simulink model "CSTR_Simulink"  (R2026a)
settings: Solver=ode15s  StopTime=model.time  FixedStep=5./60./10000
values from neighbouring files (symbols this model uses):
  A = 16.66    [plant_data_gen.m]
  Cv_Q = SS.Q ./ ( SS.lQ .* N .* sqrt( ( SS.P_U - SS.P_D ) ./ g_s) )    [plant_data_gen.m]
  Cv_Q_C = SS.Q_C ./ ( SS.lQ_C .* N .* sqrt( ( SS.P_CU - SS.P_CD ) ./ g_s ) )    [plant_data_gen.m]
  deltaH = -5e4    (= -50000)    [plant_data_gen.m]
  EoR = 8750    [plant_data_gen.m]
  g_s = 1    [plant_data_gen.m]
  K = size(x)    [PPCA_validation.m]    (also in plant_data_gen.m = 0.0625)
  k_0 = 7.2e10    (= 72000000000)    [plant_data_gen.m]
  Kc_h = -3.0    (= -3)    [plant_data_gen.m]
  Kc_Q = 0.2    [plant_data_gen.m]
  Kc_Q_C = 0.2    [plant_data_gen.m]
  Kc_T = -2.0    (= -2)    [plant_data_gen.m]
  Km_Q = 8/100    (= 0.08)    [plant_data_gen.m]
  Km_Q_C = 8/15    (= 0.533333333333)    [plant_data_gen.m]
  N = 0.0865 * 1000 / 60 / sqrt(1000)    [plant_data_gen.m]
  rhoCp = 239    [plant_data_gen.m]
  rhoCp_C = 4175    [plant_data_gen.m]
  tau = 2./60    (= 0.0333333333333)    [plant_data_gen.m]
  TI_h = 1./TI_h    (= 0.666666666667)    [plant_data_gen.m]
  TI_Q = 1.7/60    (= 0.0283333333333)    [plant_data_gen.m]
  TI_Q_C = 1./TI_Q_C    (= 35.2941176471)    [plant_data_gen.m]
  TI_T = 1./TI_T    (= 1.14942528736)    [plant_data_gen.m]
  UA_C = 5e4    (= 50000)    [plant_data_gen.m]
  V_C = 10    [plant_data_gen.m]
undefined symbols (not defined in the file or in its folder): D, model, noise, SS
libraries: dspsrcs4 x16, simulink x8, slpidlib x4
(part 1 of 2)
settings Model: Creator=danie  LastModifiedBy=daniel

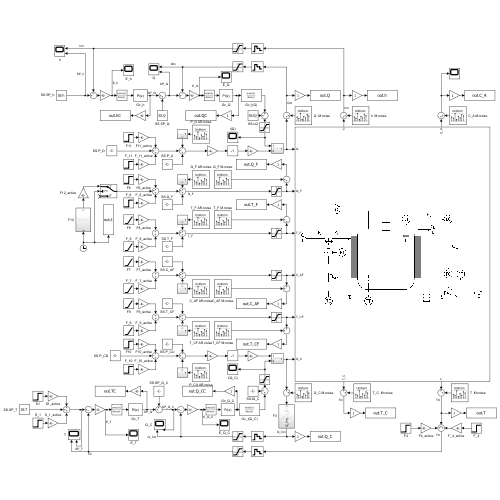
[thumbnail: Simulink's stored preview of the top-level diagram]
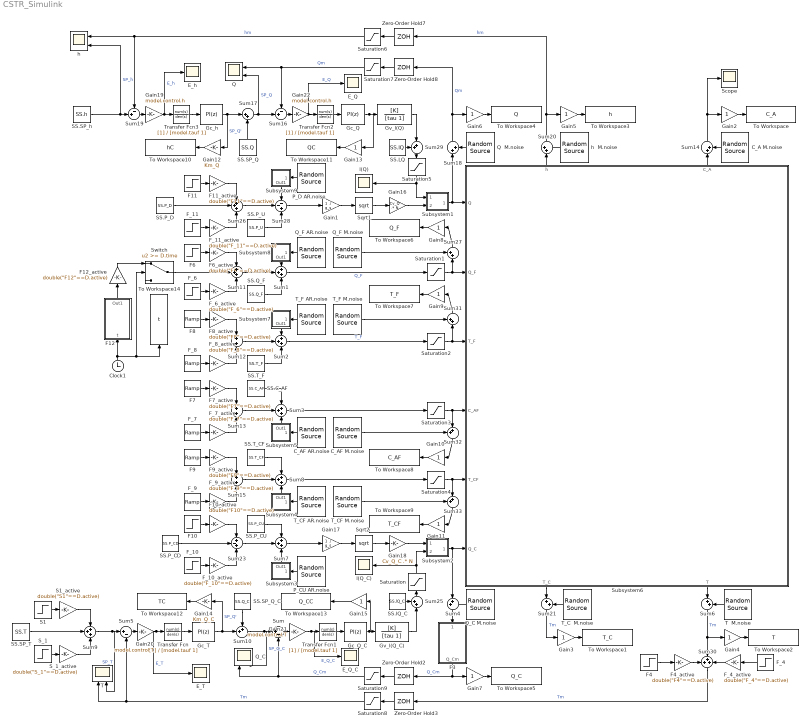
== system CSTR_Simulink ==
  C_A M.noise : dspsrcs4/Random Source  SrcType=Gaussian  MinVal=0  MaxVal=1  MeanVal=0  VarVal=noise.M.C_A.*noise.M.active  RepMode=Not repeatable  rawSeed=5  IsInherit=off  SampTime=model.dt  SampFrame=1  OutComplex=Real  DataType=double  SimulateUsing=Interpreted execution
  C_AF AR.noise : dspsrcs4/Random Source  SrcType=Gaussian  MinVal=0  MaxVal=1  MeanVal=0  VarVal=noise.AR.C_AF.*noise.AR.active  RepMode=Not repeatable  rawSeed=736  IsInherit=off  SampTime=model.dt  SampFrame=1  OutComplex=Real  DataType=double  SimulateUsing=Interpreted execution
  C_AF M.noise : dspsrcs4/Random Source  SrcType=Gaussian  MinVal=0  MaxVal=1  MeanVal=0  VarVal=noise.M.C_AF.*noise.M.active  RepMode=Not repeatable  rawSeed=3456  IsInherit=off  SampTime=model.dt  SampFrame=1  OutComplex=Real  DataType=double  SimulateUsing=Interpreted execution
  Clock1 : Clock
  E_Q : Scope
      settings: ActiveDisplayYMinimum=-115  ActiveDisplayYMaximum=135  DataLoggingVariableName=ScopeData6
  E_Q_C : Scope
      settings: ActiveDisplayYMinimum=-0.48410226680583923  ActiveDisplayYMaximum=0.37217378043200133  DataLoggingVariableName=ScopeData5
  E_T : Scope
      settings: ActiveDisplayYMinimum=-14.355250634138558  ActiveDisplayYMaximum=1.5950278482376172  DataLoggingVariableName=ScopeData4
  E_h : Scope
      settings: ActiveDisplayYMinimum=-14.355250634138558  ActiveDisplayYMaximum=1.5950278482376172  DataLoggingVariableName=ScopeData7
  F{4,6,10..11} (4 alike) : Step  Time=D.time  FinalValue=D.val  SampleTime=0
  F10_active : Gain  Gain="double(\"F10\"==D.active)"
  F11_active : Gain  Gain="double(\"F11\"==D.active)"
  F12 : Subsystem
  F12_active : Gain  Gain="double(\"F12\"==D.active)"
  F3 : Subsystem
  F4_active : Gain  Gain="double(\"F4\"==D.active)"
  F6_active : Gain  Gain="double(\"F6\"==D.active)"
  F7 : simulink/Sources/Ramp  slope=D.val  start=D.time  InitialOutput=0
  F7_active : Gain  Gain="double(\"F7\"==D.active)"
  F8 : simulink/Sources/Ramp  slope=D.val  start=D.time  InitialOutput=0
  F8_active : Gain  Gain="double(\"F8\"==D.active)"
  F9 : simulink/Sources/Ramp  slope=D.val  start=D.time  InitialOutput=0
  F9_active : Gain  Gain="double(\"F9\"==D.active)"
  F_{4,6,10..11} (4 alike) : Step  Time=D.time  FinalValue=D.val  SampleTime=0
  F_10_active : Gain  Gain="double(\"F_10\"==D.active)"
  F_11_active : Gain  Gain="double(\"F_11\"==D.active)"
  F_4_active : Gain  Gain="double(\"F_4\"==D.active)"
  F_6_active : Gain  Gain="double(\"F_6\"==D.active)"
  F_7 : simulink/Sources/Ramp  slope=D.val  start=D.time  InitialOutput=0
  F_7_active : Gain  Gain="double(\"F_7\"==D.active)"
  F_8 : simulink/Sources/Ramp  slope=D.val  start=D.time  InitialOutput=0
  F_8_active : Gain  Gain="double(\"F_8\"==D.active)"
  F_9 : simulink/Sources/Ramp  slope=D.val  start=D.time  InitialOutput=0
  F_9_active : Gain  Gain="double(\"F_9\"==D.active)"
  Gain1 : Gain  Gain=1 ./ g_s
  Gain{2..11,13,15} (12 alike) : Gain
  Gain12 : Gain  Gain=Km_Q
  Gain14 : Gain  Gain=Km_Q_C
  Gain16 : Gain  Gain=Cv_Q .* N
  Gain17 : Gain  Gain=1 ./ g_s
  Gain18 : Gain  Gain=Cv_Q_C .* N
  Gain19 : Gain  Gain=model.control.h
  Gain20 : Gain  Gain=model.control.T
  Gain21 : Gain  Gain=model.control.T
  Gain22 : Gain  Gain=model.control.h
  Gc_Q : slpidlib/PID Controller  Controller=PI  Form=Ideal  TimeDomain=Discrete-time  UseExternalTs=off  SampleTime=model.dt  IntegratorMethod=Forward Euler  FilterMethod=Forward Euler  ControllerParametersSource=internal  P=Kc_Q  I=TI_Q  UseKiTs=off  D=0  UseExternalDerivativeSource=off  N=100  UseFilter=on  TunerSelectOption=Transfer Function Based (PID Tuner App)  InitialConditionSource=internal  InitialConditionForIntegrator=0  InitialConditionForFilter=0  DifferentiatorICPrevScaledInput=0  ExternalReset=none  TrackingMode=off  Kt=1  LimitOutput=off  SatLimitsSource=internal  UpperSaturationLimit=inf  LowerSaturationLimit=-inf  LinearizeAsGain=on  AntiWindupMode=none  Kb=1  LimitIntegrator=off  UpperIntegratorSaturationLimit=inf  LowerIntegratorSaturationLimit=-inf  POutMin=[]  POutMax=[]  IOutMin=[]  IOutMax=[]  DOutMin=[]  DOutMax=[]  NOutMin=[]  NOutMax=[]  SumOutMin=[]  SumOutMax=[]  SaturationOutMin=[]  SaturationOutMax=[]  PParamMin=[]  PParamMax=[]  IParamMin=[]  IParamMax=[]  DParamMin=[]  DParamMax=[]  NParamMin=[]  NParamMax=[]  KbParamMin=[]  KbParamMax=[]  KtParamMin=[]  KtParamMax=[]  KbOutMin=[]  KbOutMax=[]  KtOutMin=[]  KtOutMax=[]  IntegratorOutMin=[]  IntegratorOutMax=[]  FilterOutMin=[]  FilterOutMax=[]  SumI1OutMin=[]  SumI1OutMax=[]  SumI2OutMin=[]  SumI2OutMax=[]  SumI3OutMin=[]  SumI3OutMax=[]  SumI4OutMin=[]  SumI4OutMax=[]  SumDOutMin=[]  SumDOutMax=[]  DifferentiatorOutMin=[]  DifferentiatorOutMax=[]  FilterDiffOutCoefMin=[]  FilterDiffOutCoefMax=[]  ReciprocalOutMin=[]  ReciprocalOutMax=[]  SumDenOutMin=[]  SumDenOutMax=[]  SumNumOutMin=[]  SumNumOutMax=[]  DivideOutMin=[]  DivideOutMax=[]  UdiffTsProdOutMin=[]  UdiffTsProdOutMax=[]  NTsProdOutMin=[]  NTsProdOutMax=[]  UintegralTsProdOutMin=[]  UintegralTsProdOutMax=[]  UngainTsProdOutMin=[]  UngainTsProdOutMax=[]  ClampingZeroOutDataTypeStr=Inherit: Inherit via back propagation  ClampingZeroOutMin=[]  ClampingZeroOutMax=[]  FilterDenConstantOutDataTypeStr=Inherit: Inherit via back propagation  FilterDenConstantOutMin=[]  FilterDenConstantOutMax=[]  PCopyOutDataTypeStr=Inherit: Inherit via back propagation  PCopyOutMin=[]  PCopyOutMax=[]  NCopyOutDataTypeStr=Inherit: Inherit via back propagation  NCopyOutMin=[]  NCopyOutMax=[]  IntegratorContinuousStateAttributes=''  IntegratorStateMustResolveToSignalObject=off  IntegratorRTWStateStorageClass=Auto  FilterContinuousStateAttributes=''  FilterStateMustResolveToSignalObject=off  FilterRTWStateStorageClass=Auto  ParallelPVariant=Passthrough  IdealPVariant=InternalParameters  IVariant=InternalParameters  DVariant=Disabled  IntegratorVariant=Discrete  SatVariant=Disabled  AWVariant=Passthrough  PCopyVariant=Disabled  TRVariant=Disabled  FdbkBlocksVariant=Forward  IdealPFdbkVariant=Disabled  SatFdbkVariant=Disabled  DerivativeFilterVariant=Disabled  NVariant=Disabled  NCopyVariant=Disabled_SignalSpec  FilterICVariant=Disabled  IntegratorICVariant=InternalICs  ExternalResetVariant=Disabled  TRSumVariant=Passthrough  SumFdbkVariant=Disabled  SumVariant=Sum_PI  TsampFilterVariant=InternalTs  TsampNgainVariant=Passthrough  TsampIntegralVariant=Disabled_SignalSpec  ExternalSaturationOutDataTypeStr=Inherit: Same as second input  DerivativeSourceVariant=Disabled  PreIntVariant=InternalPreInt
  Gc_Q_C : slpidlib/PID Controller  Controller=PI  Form=Ideal  TimeDomain=Discrete-time  UseExternalTs=off  SampleTime=model.dt  IntegratorMethod=Forward Euler  FilterMethod=Forward Euler  ControllerParametersSource=internal  P=Kc_Q_C  I=TI_Q_C  UseKiTs=off  D=0  UseExternalDerivativeSource=off  N=100  UseFilter=on  TunerSelectOption=Transfer Function Based (PID Tuner App)  InitialConditionSource=internal  InitialConditionForIntegrator=0  InitialConditionForFilter=0  DifferentiatorICPrevScaledInput=0  ExternalReset=none  TrackingMode=off  Kt=1  LimitOutput=off  SatLimitsSource=internal  UpperSaturationLimit=inf  LowerSaturationLimit=-inf  LinearizeAsGain=on  AntiWindupMode=none  Kb=1  LimitIntegrator=off  UpperIntegratorSaturationLimit=inf  LowerIntegratorSaturationLimit=-inf  POutMin=[]  POutMax=[]  IOutMin=[]  IOutMax=[]  DOutMin=[]  DOutMax=[]  NOutMin=[]  NOutMax=[]  SumOutMin=[]  SumOutMax=[]  SaturationOutMin=[]  SaturationOutMax=[]  PParamMin=[]  PParamMax=[]  IParamMin=[]  IParamMax=[]  DParamMin=[]  DParamMax=[]  NParamMin=[]  NParamMax=[]  KbParamMin=[]  KbParamMax=[]  KtParamMin=[]  KtParamMax=[]  KbOutMin=[]  KbOutMax=[]  KtOutMin=[]  KtOutMax=[]  IntegratorOutMin=[]  IntegratorOutMax=[]  FilterOutMin=[]  FilterOutMax=[]  SumI1OutMin=[]  SumI1OutMax=[]  SumI2OutMin=[]  SumI2OutMax=[]  SumI3OutMin=[]  SumI3OutMax=[]  SumI4OutMin=[]  SumI4OutMax=[]  SumDOutMin=[]  SumDOutMax=[]  DifferentiatorOutMin=[]  DifferentiatorOutMax=[]  FilterDiffOutCoefMin=[]  FilterDiffOutCoefMax=[]  ReciprocalOutMin=[]  ReciprocalOutMax=[]  SumDenOutMin=[]  SumDenOutMax=[]  SumNumOutMin=[]  SumNumOutMax=[]  DivideOutMin=[]  DivideOutMax=[]  UdiffTsProdOutMin=[]  UdiffTsProdOutMax=[]  NTsProdOutMin=[]  NTsProdOutMax=[]  UintegralTsProdOutMin=[]  UintegralTsProdOutMax=[]  UngainTsProdOutMin=[]  UngainTsProdOutMax=[]  ClampingZeroOutDataTypeStr=Inherit: Inherit via back propagation  ClampingZeroOutMin=[]  ClampingZeroOutMax=[]  FilterDenConstantOutDataTypeStr=Inherit: Inherit via back propagation  FilterDenConstantOutMin=[]  FilterDenConstantOutMax=[]  PCopyOutDataTypeStr=Inherit: Inherit via back propagation  PCopyOutMin=[]  PCopyOutMax=[]  NCopyOutDataTypeStr=Inherit: Inherit via back propagation  NCopyOutMin=[]  NCopyOutMax=[]  IntegratorContinuousStateAttributes=''  IntegratorStateMustResolveToSignalObject=off  IntegratorRTWStateStorageClass=Auto  FilterContinuousStateAttributes=''  FilterStateMustResolveToSignalObject=off  FilterRTWStateStorageClass=Auto  ParallelPVariant=Passthrough  IdealPVariant=InternalParameters  IVariant=InternalParameters  DVariant=Disabled  IntegratorVariant=Discrete  SatVariant=Disabled  AWVariant=Passthrough  PCopyVariant=Disabled  TRVariant=Disabled  FdbkBlocksVariant=Forward  IdealPFdbkVariant=Disabled  SatFdbkVariant=Disabled  DerivativeFilterVariant=Disabled  NVariant=Disabled  NCopyVariant=Disabled_SignalSpec  FilterICVariant=Disabled  IntegratorICVariant=InternalICs  ExternalResetVariant=Disabled  TRSumVariant=Passthrough  SumFdbkVariant=Disabled  SumVariant=Sum_PI  TsampFilterVariant=InternalTs  TsampNgainVariant=Passthrough  TsampIntegralVariant=Disabled_SignalSpec  ExternalSaturationOutDataTypeStr=Inherit: Same as second input  DerivativeSourceVariant=Disabled  PreIntVariant=InternalPreInt
  Gc_T : slpidlib/PID Controller  Controller=PI  Form=Ideal  TimeDomain=Discrete-time  UseExternalTs=off  SampleTime=model.dt  IntegratorMethod=Forward Euler  FilterMethod=Forward Euler  ControllerParametersSource=internal  P=Kc_T  I=TI_T  UseKiTs=off  D=0  UseExternalDerivativeSource=off  N=100  UseFilter=on  TunerSelectOption=Transfer Function Based (PID Tuner App)  InitialConditionSource=internal  InitialConditionForIntegrator=0  InitialConditionForFilter=0  DifferentiatorICPrevScaledInput=0  ExternalReset=none  TrackingMode=off  Kt=1  LimitOutput=off  SatLimitsSource=internal  UpperSaturationLimit=inf  LowerSaturationLimit=-inf  LinearizeAsGain=on  AntiWindupMode=none  Kb=1  LimitIntegrator=off  UpperIntegratorSaturationLimit=inf  LowerIntegratorSaturationLimit=-inf  POutMin=[]  POutMax=[]  IOutMin=[]  IOutMax=[]  DOutMin=[]  DOutMax=[]  NOutMin=[]  NOutMax=[]  SumOutMin=[]  SumOutMax=[]  SaturationOutMin=[]  SaturationOutMax=[]  PParamMin=[]  PParamMax=[]  IParamMin=[]  IParamMax=[]  DParamMin=[]  DParamMax=[]  NParamMin=[]  NParamMax=[]  KbParamMin=[]  KbParamMax=[]  KtParamMin=[]  KtParamMax=[]  KbOutMin=[]  KbOutMax=[]  KtOutMin=[]  KtOutMax=[]  IntegratorOutMin=[]  IntegratorOutMax=[]  FilterOutMin=[]  FilterOutMax=[]  SumI1OutMin=[]  SumI1OutMax=[]  SumI2OutMin=[]  SumI2OutMax=[]  SumI3OutMin=[]  SumI3OutMax=[]  SumI4OutMin=[]  SumI4OutMax=[]  SumDOutMin=[]  SumDOutMax=[]  DifferentiatorOutMin=[]  DifferentiatorOutMax=[]  FilterDiffOutCoefMin=[]  FilterDiffOutCoefMax=[]  ReciprocalOutMin=[]  ReciprocalOutMax=[]  SumDenOutMin=[]  SumDenOutMax=[]  SumNumOutMin=[]  SumNumOutMax=[]  DivideOutMin=[]  DivideOutMax=[]  UdiffTsProdOutMin=[]  UdiffTsProdOutMax=[]  NTsProdOutMin=[]  NTsProdOutMax=[]  UintegralTsProdOutMin=[]  UintegralTsProdOutMax=[]  UngainTsProdOutMin=[]  UngainTsProdOutMax=[]  ClampingZeroOutDataTypeStr=Inherit: Inherit via back propagation  ClampingZeroOutMin=[]  ClampingZeroOutMax=[]  FilterDenConstantOutDataTypeStr=Inherit: Inherit via back propagation  FilterDenConstantOutMin=[]  FilterDenConstantOutMax=[]  PCopyOutDataTypeStr=Inherit: Inherit via back propagation  PCopyOutMin=[]  PCopyOutMax=[]  NCopyOutDataTypeStr=Inherit: Inherit via back propagation  NCopyOutMin=[]  NCopyOutMax=[]  IntegratorContinuousStateAttributes=''  IntegratorStateMustResolveToSignalObject=off  IntegratorRTWStateStorageClass=Auto  FilterContinuousStateAttributes=''  FilterStateMustResolveToSignalObject=off  FilterRTWStateStorageClass=Auto  ParallelPVariant=Passthrough  IdealPVariant=InternalParameters  IVariant=InternalParameters  DVariant=Disabled  IntegratorVariant=Discrete  SatVariant=Disabled  AWVariant=Passthrough  PCopyVariant=Disabled  TRVariant=Disabled  FdbkBlocksVariant=Forward  IdealPFdbkVariant=Disabled  SatFdbkVariant=Disabled  DerivativeFilterVariant=Disabled  NVariant=Disabled  NCopyVariant=Disabled_SignalSpec  FilterICVariant=Disabled  IntegratorICVariant=InternalICs  ExternalResetVariant=Disabled  TRSumVariant=Passthrough  SumFdbkVariant=Disabled  SumVariant=Sum_PI  TsampFilterVariant=InternalTs  TsampNgainVariant=Passthrough  TsampIntegralVariant=Disabled_SignalSpec  ExternalSaturationOutDataTypeStr=Inherit: Same as second input  DerivativeSourceVariant=Disabled  PreIntVariant=InternalPreInt
  Gc_h : slpidlib/PID Controller  Controller=PI  Form=Ideal  TimeDomain=Discrete-time  UseExternalTs=off  SampleTime=model.dt  IntegratorMethod=Forward Euler  FilterMethod=Forward Euler  ControllerParametersSource=internal  P=Kc_h  I=TI_h  UseKiTs=off  D=0  UseExternalDerivativeSource=off  N=100  UseFilter=on  TunerSelectOption=Transfer Function Based (PID Tuner App)  InitialConditionSource=internal  InitialConditionForIntegrator=0  InitialConditionForFilter=0  DifferentiatorICPrevScaledInput=0  ExternalReset=none  TrackingMode=off  Kt=1  LimitOutput=off  SatLimitsSource=internal  UpperSaturationLimit=inf  LowerSaturationLimit=-inf  LinearizeAsGain=on  AntiWindupMode=none  Kb=1  LimitIntegrator=off  UpperIntegratorSaturationLimit=inf  LowerIntegratorSaturationLimit=-inf  POutMin=[]  POutMax=[]  IOutMin=[]  IOutMax=[]  DOutMin=[]  DOutMax=[]  NOutMin=[]  NOutMax=[]  SumOutMin=[]  SumOutMax=[]  SaturationOutMin=[]  SaturationOutMax=[]  PParamMin=[]  PParamMax=[]  IParamMin=[]  IParamMax=[]  DParamMin=[]  DParamMax=[]  NParamMin=[]  NParamMax=[]  KbParamMin=[]  KbParamMax=[]  KtParamMin=[]  KtParamMax=[]  KbOutMin=[]  KbOutMax=[]  KtOutMin=[]  KtOutMax=[]  IntegratorOutMin=[]  IntegratorOutMax=[]  FilterOutMin=[]  FilterOutMax=[]  SumI1OutMin=[]  SumI1OutMax=[]  SumI2OutMin=[]  SumI2OutMax=[]  SumI3OutMin=[]  SumI3OutMax=[]  SumI4OutMin=[]  SumI4OutMax=[]  SumDOutMin=[]  SumDOutMax=[]  DifferentiatorOutMin=[]  DifferentiatorOutMax=[]  FilterDiffOutCoefMin=[]  FilterDiffOutCoefMax=[]  ReciprocalOutMin=[]  ReciprocalOutMax=[]  SumDenOutMin=[]  SumDenOutMax=[]  SumNumOutMin=[]  SumNumOutMax=[]  DivideOutMin=[]  DivideOutMax=[]  UdiffTsProdOutMin=[]  UdiffTsProdOutMax=[]  NTsProdOutMin=[]  NTsProdOutMax=[]  UintegralTsProdOutMin=[]  UintegralTsProdOutMax=[]  UngainTsProdOutMin=[]  UngainTsProdOutMax=[]  ClampingZeroOutDataTypeStr=Inherit: Inherit via back propagation  ClampingZeroOutMin=[]  ClampingZeroOutMax=[]  FilterDenConstantOutDataTypeStr=Inherit: Inherit via back propagation  FilterDenConstantOutMin=[]  FilterDenConstantOutMax=[]  PCopyOutDataTypeStr=Inherit: Inherit via back propagation  PCopyOutMin=[]  PCopyOutMax=[]  NCopyOutDataTypeStr=Inherit: Inherit via back propagation  NCopyOutMin=[]  NCopyOutMax=[]  IntegratorContinuousStateAttributes=''  IntegratorStateMustResolveToSignalObject=off  IntegratorRTWStateStorageClass=Auto  FilterContinuousStateAttributes=''  FilterStateMustResolveToSignalObject=off  FilterRTWStateStorageClass=Auto  ParallelPVariant=Passthrough  IdealPVariant=InternalParameters  IVariant=InternalParameters  DVariant=Disabled  IntegratorVariant=Discrete  SatVariant=Disabled  AWVariant=Passthrough  PCopyVariant=Disabled  TRVariant=Disabled  FdbkBlocksVariant=Forward  IdealPFdbkVariant=Disabled  SatFdbkVariant=Disabled  DerivativeFilterVariant=Disabled  NVariant=Disabled  NCopyVariant=Disabled_SignalSpec  FilterICVariant=Disabled  IntegratorICVariant=InternalICs  ExternalResetVariant=Disabled  TRSumVariant=Passthrough  SumFdbkVariant=Disabled  SumVariant=Sum_PI  TsampFilterVariant=InternalTs  TsampNgainVariant=Passthrough  TsampIntegralVariant=Disabled_SignalSpec  ExternalSaturationOutDataTypeStr=Inherit: Same as second input  DerivativeSourceVariant=Disabled  PreIntVariant=InternalPreInt
  Gv_l(Q) : TransferFcn  Numerator=[K]  Denominator=[tau 1]
  Gv_l(Q_C) : TransferFcn  Numerator=[K]  Denominator=[tau 1]
  P_CU AR.noise : dspsrcs4/Random Source  SrcType=Gaussian  MinVal=0  MaxVal=1  MeanVal=0  VarVal=noise.AR.P_CU.*noise.AR.active  RepMode=Not repeatable  rawSeed=67  IsInherit=off  SampTime=model.dt  SampFrame=1  OutComplex=Real  DataType=double  SimulateUsing=Interpreted execution
  P_D AR.noise : dspsrcs4/Random Source  SrcType=Gaussian  MinVal=0  MaxVal=1  MeanVal=0  VarVal=noise.AR.P_D.*noise.AR.active  RepMode=Not repeatable  rawSeed=92  IsInherit=off  SampTime=model.dt  SampFrame=1  OutComplex=Real  DataType=double  SimulateUsing=Interpreted execution
  Q : Scope  NumInputPorts=2
      settings: SampleTime=5/60  ActiveDisplayYMinimum=-1.5483487022841418  ActiveDisplayYMaximum=201.98285760431011  DataLoggingVariableName=ScopeData8
  Q  M.noise : dspsrcs4/Random Source  SrcType=Gaussian  MinVal=0  MaxVal=1  MeanVal=0  VarVal=noise.M.Q.*noise.M.active  RepMode=Not repeatable  rawSeed=23  IsInherit=off  SampTime=model.dt  SampFrame=1  OutComplex=Real  DataType=double  SimulateUsing=Interpreted execution
  Q_C : Scope  NumInputPorts=2
      settings: SampleTime=5/60  ActiveDisplayYMinimum=14.627826219567998  ActiveDisplayYMaximum=15.484102266805841  DataLoggingVariableName=ScopeData10
  Q_C M.noise : dspsrcs4/Random Source  SrcType=Gaussian  MinVal=0  MaxVal=1  MeanVal=0  VarVal=noise.M.Q_C.*noise.M.active  RepMode=Not repeatable  rawSeed=3  IsInherit=off  SampTime=model.dt  SampFrame=1  OutComplex=Real  DataType=double  SimulateUsing=Interpreted execution
  Q_F AR.noise : dspsrcs4/Random Source  SrcType=Gaussian  MinVal=0  MaxVal=1  MeanVal=0  VarVal=noise.AR.Q_F.*noise.AR.active  RepMode=Not repeatable  rawSeed=104  IsInherit=off  SampTime=model.dt  SampFrame=1  OutComplex=Real  DataType=double  SimulateUsing=Interpreted execution
  Q_F M.noise : dspsrcs4/Random Source  SrcType=Gaussian  MinVal=0  MaxVal=1  MeanVal=0  VarVal=noise.M.Q_F.*noise.M.active  RepMode=Not repeatable  rawSeed=5467  IsInherit=off  SampTime=model.dt  SampFrame=1  OutComplex=Real  DataType=double  SimulateUsing=Interpreted execution
  S1 : Step  Time=D.time  FinalValue=D.val  SampleTime=0
  S1_active : Gain  Gain="double(\"S1\"==D.active)"
  SS.C_AF : Constant  Value=SS.C_AF
  SS.LQ : Constant  Value=SS.lQ
  SS.P_CD : Constant  Value=SS.P_CD
  SS.P_CU : Constant  Value=SS.P_CU
  SS.P_D : Constant  Value=SS.P_D
  SS.P_U : Constant  Value=SS.P_U
  SS.Q_F : Constant  Value=SS.Q_F
  SS.SP_Q : Constant  Value=SS.Q
  SS.SP_Q_C : Constant  Value=SS.Q_C
  SS.SP_T : Constant  Value=SS.T
  SS.SP_h : Constant  Value=SS.h
  SS.T_CF : Constant  Value=SS.T_CF
  SS.T_F : Constant  Value=SS.T_F
  SS.lQ_C : Constant  Value=SS.lQ_C
  S_1 : Step  Time=D.time  FinalValue=D.val  SampleTime=0
  S_1_active : Gain  Gain="double(\"S_1\"==D.active)"
  Saturation : Saturate  UpperLimit=1  LowerLimit=0
  Saturation{1..4} (4 alike) : Saturate  UpperLimit=Inf  LowerLimit=0
  Saturation5 : Saturate  UpperLimit=1  LowerLimit=0
  Saturation{6..9} (4 alike) : Saturate  UpperLimit=inf  LowerLimit=0
  Scope : Scope
      settings: ActiveDisplayYMinimum=-1  ActiveDisplayYMaximum=1
  Sqrt1 : Sqrt
  Sqrt2 : Sqrt
  Subsystem1 : Subsystem
  Subsystem2 : Subsystem
  Subsystem3 : Subsystem
      settings: PortSchema="{\"entries\":[{\"content\":{\"sides\":[{\"content\":{},\"type\":\"ConnectorPlacement.EquallySpacedRectSide\",\"uuid\":\"f496c22c-98f8-4657-b261-2f509f1099bb\"},{\"content\":{\"connectorIds\":[\"In1\"],\"side\":\"RIGHT\"},\"type\":\"ConnectorPlacement.EquallySpacedRectSide\",\"uuid\":\"54c2bc8d-f04e-48ab-99ca-70382f6eea1e\"},{\"content\":{\"connectorIds\":[\"Out1\"],\"side\":\"TOP\"},\"type\":\"ConnectorPlacement.EquallySpacedRectSide\",\"uuid\":\"161c4006-1b8b-4a02-9971-04e72c9ff37a\"}]},\"type\":\"ConnectorPlacement.EquallySpacedConnector\",\"uuid\":\"f38e24fa-e926-432e-ab74-a548c7cce3b1\"}],\"packageUris\":[\"http://schema.mathworks.com/mf0/Connector/R2020b\"],\"version\":\"1.0\"}"
  Subsystem4 : Subsystem
      settings: PortSchema="{\"entries\":[{\"content\":{\"sides\":[{\"content\":{},\"type\":\"ConnectorPlacement.EquallySpacedRectSide\",\"uuid\":\"f496c22c-98f8-4657-b261-2f509f1099bb\"},{\"content\":{\"connectorIds\":[\"In1\"],\"side\":\"RIGHT\"},\"type\":\"ConnectorPlacement.EquallySpacedRectSide\",\"uuid\":\"54c2bc8d-f04e-48ab-99ca-70382f6eea1e\"},{\"content\":{\"connectorIds\":[\"Out1\"],\"side\":\"TOP\"},\"type\":\"ConnectorPlacement.EquallySpacedRectSide\",\"uuid\":\"161c4006-1b8b-4a02-9971-04e72c9ff37a\"}]},\"type\":\"ConnectorPlacement.EquallySpacedConnector\",\"uuid\":\"f38e24fa-e926-432e-ab74-a548c7cce3b1\"}],\"packageUris\":[\"http://schema.mathworks.com/mf0/Connector/R2020b\"],\"version\":\"1.0\"}"
  Subsystem5 : Subsystem
      settings: PortSchema="{\"entries\":[{\"content\":{\"sides\":[{\"content\":{},\"type\":\"ConnectorPlacement.EquallySpacedRectSide\",\"uuid\":\"f496c22c-98f8-4657-b261-2f509f1099bb\"},{\"content\":{\"connectorIds\":[\"In1\"],\"side\":\"RIGHT\"},\"type\":\"ConnectorPlacement.EquallySpacedRectSide\",\"uuid\":\"54c2bc8d-f04e-48ab-99ca-70382f6eea1e\"},{\"content\":{\"connectorIds\":[\"Out1\"],\"side\":\"TOP\"},\"type\":\"ConnectorPlacement.EquallySpacedRectSide\",\"uuid\":\"161c4006-1b8b-4a02-9971-04e72c9ff37a\"}]},\"type\":\"ConnectorPlacement.EquallySpacedConnector\",\"uuid\":\"f38e24fa-e926-432e-ab74-a548c7cce3b1\"}],\"packageUris\":[\"http://schema.mathworks.com/mf0/Connector/R2020b\"],\"version\":\"1.0\"}"
  Subsystem6 : Subsystem
      settings: PortSchema="{\"entries\":[{\"content\":{\"sides\":[{\"content\":{\"connectorIds\":[\"In1\",\"In2\",\"In3\",\"In4\",\"In5\",\"In6\"]},\"type\":\"ConnectorPlacement.EquallySpacedRectSide\",\"uuid\":\"337e4d9c-e607-49c3-9a51-810a8ea00862\"},{\"content\":{\"side\":\"RIGHT\"},\"type\":\"ConnectorPlacement.EquallySpacedRectSide\",\"uuid\":\"44cb8c56-a8c0-4416-aa4b-008addea6ed1\"},{\"content\":{\"connectorIds\":[\"Out3\",\"Out4\"],\"side\":\"TOP\"},\"type\":\"ConnectorPlacement.EquallySpacedRectSide\",\"uuid\":\"6424ee35-6e69-4da1-a80e-4d7ee51c02b7\"},{\"content\":{\"connectorIds\":[\"Out1\",\"Out2\"],\"side\":\"BOTTOM\"},\"type\":\"ConnectorPlacement.EquallySpacedRectSide\",\"uuid\":\"b6ba0e0a-8754-4e64-a604-c52ee032ea64\"}]},\"type\":\"ConnectorPlacement.EquallySpacedConnector\",\"uuid\":\"3a5123cf-2c87-4d93-ac46-895c86de09ce\"}],\"packageUris\":[\"http://schema.mathworks.com/mf0/Connector/R2020b\"],\"version\":\"1.0\"}"
      mask Display: image('CSTR_figure.png', [0,0,0,0,100,75]);
  Subsystem7 : Subsystem
      settings: PortSchema="{\"entries\":[{\"content\":{\"sides\":[{\"content\":{},\"type\":\"ConnectorPlacement.EquallySpacedRectSide\",\"uuid\":\"f496c22c-98f8-4657-b261-2f509f1099bb\"},{\"content\":{\"connectorIds\":[\"In1\"],\"side\":\"RIGHT\"},\"type\":\"ConnectorPlacement.EquallySpacedRectSide\",\"uuid\":\"54c2bc8d-f04e-48ab-99ca-70382f6eea1e\"},{\"content\":{\"side\":\"TOP\"},\"type\":\"ConnectorPlacement.EquallySpacedRectSide\",\"uuid\":\"161c4006-1b8b-4a02-9971-04e72c9ff37a\"},{\"content\":{\"connectorIds\":[\"Out1\"],\"side\":\"BOTTOM\"},\"type\":\"ConnectorPlacement.EquallySpacedRectSide\",\"uuid\":\"4c2f02a0-dbff-4ebd-9757-86efb1809e35\"}]},\"type\":\"ConnectorPlacement.EquallySpacedConnector\",\"uuid\":\"f38e24fa-e926-432e-ab74-a548c7cce3b1\"}],\"packageUris\":[\"http://schema.mathworks.com/mf0/Connector/R2020b\"],\"version\":\"1.0\"}"
  Subsystem8 : Subsystem
      settings: PortSchema="{\"entries\":[{\"content\":{\"sides\":[{\"content\":{},\"type\":\"ConnectorPlacement.EquallySpacedRectSide\",\"uuid\":\"f496c22c-98f8-4657-b261-2f509f1099bb\"},{\"content\":{\"connectorIds\":[\"In1\"],\"side\":\"RIGHT\"},\"type\":\"ConnectorPlacement.EquallySpacedRectSide\",\"uuid\":\"54c2bc8d-f04e-48ab-99ca-70382f6eea1e\"},{\"content\":{\"side\":\"TOP\"},\"type\":\"ConnectorPlacement.EquallySpacedRectSide\",\"uuid\":\"161c4006-1b8b-4a02-9971-04e72c9ff37a\"},{\"content\":{\"connectorIds\":[\"Out1\"],\"side\":\"BOTTOM\"},\"type\":\"ConnectorPlacement.EquallySpacedRectSide\",\"uuid\":\"b294b6cc-e047-4265-ac40-f94500c16fa5\"}]},\"type\":\"ConnectorPlacement.EquallySpacedConnector\",\"uuid\":\"f38e24fa-e926-432e-ab74-a548c7cce3b1\"}],\"packageUris\":[\"http://schema.mathworks.com/mf0/Connector/R2020b\"],\"version\":\"1.0\"}"
  Subsystem9 : Subsystem
      settings: PortSchema="{\"entries\":[{\"content\":{\"sides\":[{\"content\":{\"connectorIds\":[\"In1\"]},\"type\":\"ConnectorPlacement.EquallySpacedRectSide\",\"uuid\":\"c8e993dd-d0ed-40c8-9029-0d750a843fbf\"},{\"content\":{\"side\":\"RIGHT\"},\"type\":\"ConnectorPlacement.EquallySpacedRectSide\",\"uuid\":\"0fc18147-112d-4800-9543-a03be0484f31\"},{\"content\":{\"side\":\"TOP\"},\"type\":\"ConnectorPlacement.EquallySpacedRectSide\",\"uuid\":\"4960ba26-b990-407b-bb70-0935e6528d79\"},{\"content\":{\"connectorIds\":[\"Out1\"],\"side\":\"BOTTOM\"},\"type\":\"ConnectorPlacement.EquallySpacedRectSide\",\"uuid\":\"dbd71705-215c-4fea-82d9-9d69185a3396\"}]},\"type\":\"ConnectorPlacement.EquallySpacedConnector\",\"uuid\":\"1a1d1c9a-ca63-40d6-aa06-81c81052c4c4\"}],\"packageUris\":[\"http://schema.mathworks.com/mf0/Connector/R2020b\"],\"version\":\"1.0\"}"
  Sum : Sum  Inputs=|+-
  Sum{1..3,7..9,11,26,30} (9 alike) : Sum  Inputs=+++
  Sum{10,25,27,29,31..33} (7 alike) : Sum  Inputs=++|
  Sum12 : Sum  Inputs=+|+
  Sum13 : Sum  Inputs=+|+
  Sum{4,6,14,17..18,20..21} (7 alike) : Sum  Inputs=|++
  Sum15 : Sum  Inputs=+|+
  Sum16 : Sum  Inputs=-+|
  Sum19 : Sum  Inputs=-+|
  Sum23 : Sum  Inputs=+-+
  Sum28 : Sum  Inputs=--+
  Sum5 : Sum  Inputs=|+-
  Switch : Switch  Threshold=D.time  SaturateOnIntegerOverflow=off  InputSameDT=off
  T : Scope  NumInputPorts=2
      settings: SampleTime=5/60  ActiveDisplayYMinimum=368.38027198741213  ActiveDisplayYMaximum=447.15135916556511
  T  M.noise : dspsrcs4/Random Source  SrcType=Gaussian  MinVal=0  MaxVal=1  MeanVal=0  VarVal=noise.M.T.*noise.M.active  RepMode=Not repeatable  rawSeed=6  IsInherit=off  SampTime=model.dt  SampFrame=1  OutComplex=Real  DataType=double  SimulateUsing=Interpreted execution
  T_C  M.noise : dspsrcs4/Random Source  SrcType=Gaussian  MinVal=0  MaxVal=1  MeanVal=0  VarVal=noise.M.T_C.*noise.M.active  RepMode=Not repeatable  rawSeed=6  IsInherit=off  SampTime=model.dt  SampFrame=1  OutComplex=Real  DataType=double  SimulateUsing=Interpreted execution
  T_CF AR.noise : dspsrcs4/Random Source  SrcType=Gaussian  MinVal=0  MaxVal=1  MeanVal=0  VarVal=noise.AR.T_CF.*noise.AR.active  RepMode=Not repeatable  rawSeed=21  IsInherit=off  SampTime=model.dt  SampFrame=1  OutComplex=Real  DataType=double  SimulateUsing=Interpreted execution
  T_CF M.noise : dspsrcs4/Random Source  SrcType=Gaussian  MinVal=0  MaxVal=1  MeanVal=0  VarVal=noise.M.T_CF.*noise.M.active  RepMode=Not repeatable  rawSeed=2349  IsInherit=off  SampTime=model.dt  SampFrame=1  OutComplex=Real  DataType=double  SimulateUsing=Interpreted execution
  T_F AR.noise : dspsrcs4/Random Source  SrcType=Gaussian  MinVal=0  MaxVal=1  MeanVal=0  VarVal=noise.AR.T_F.*noise.AR.active  RepMode=Not repeatable  rawSeed=57  IsInherit=off  SampTime=model.dt  SampFrame=1  OutComplex=Real  DataType=double  SimulateUsing=Interpreted execution
  T_F M.noise : dspsrcs4/Random Source  SrcType=Gaussian  MinVal=0  MaxVal=1  MeanVal=0  VarVal=noise.M.T_F.*noise.M.active  RepMode=Not repeatable  rawSeed=983  IsInherit=off  SampTime=model.dt  SampFrame=1  OutComplex=Real  DataType=double  SimulateUsing=Interpreted execution
  To Workspace : ToWorkspace  VariableName=C_A  SampleTime=model.dt
      settings: Save2DSignal=2-D array (concatenate along first dimension)
  To Workspace1 : ToWorkspace  VariableName=T_C  SampleTime=model.dt
      settings: Save2DSignal=2-D array (concatenate along first dimension)
  To Workspace10 : ToWorkspace  VariableName=hC  SampleTime=model.dt
      settings: Save2DSignal=2-D array (concatenate along first dimension)
  To Workspace11 : ToWorkspace  VariableName=QC  SampleTime=model.dt
      settings: Save2DSignal=2-D array (concatenate along first dimension)
  To Workspace12 : ToWorkspace  VariableName=TC  SampleTime=model.dt
      settings: Save2DSignal=2-D array (concatenate along first dimension)
  To Workspace13 : ToWorkspace  VariableName=Q_CC  SampleTime=model.dt
      settings: Save2DSignal=2-D array (concatenate along first dimension)
  To Workspace14 : ToWorkspace  VariableName=t  SampleTime=model.dt
      settings: Save2DSignal=2-D array (concatenate along first dimension)
  To Workspace2 : ToWorkspace  VariableName=T  SampleTime=model.dt
      settings: Save2DSignal=2-D array (concatenate along first dimension)
  To Workspace3 : ToWorkspace  VariableName=h  SampleTime=model.dt
      settings: Save2DSignal=2-D array (concatenate along first dimension)
  To Workspace4 : ToWorkspace  VariableName=Q  SampleTime=model.dt
      settings: Save2DSignal=2-D array (concatenate along first dimension)
  To Workspace5 : ToWorkspace  VariableName=Q_C  SampleTime=model.dt
      settings: Save2DSignal=2-D array (concatenate along first dimension)
  To Workspace6 : ToWorkspace  VariableName=Q_F  SampleTime=model.dt
      settings: Save2DSignal=2-D array (concatenate along first dimension)
  To Workspace7 : ToWorkspace  VariableName=T_F  SampleTime=model.dt
      settings: Save2DSignal=2-D array (concatenate along first dimension)
  To Workspace8 : ToWorkspace  VariableName=C_AF  SampleTime=model.dt
      settings: Save2DSignal=2-D array (concatenate along first dimension)
  To Workspace9 : ToWorkspace  VariableName=T_CF  SampleTime=model.dt
      settings: Save2DSignal=2-D array (concatenate along first dimension)
  Transfer Fcn{,1..3} (4 alike) : TransferFcn  Denominator=[model.tauf 1]
  Zero-Order Hold{2..3,7..8} (4 alike) : ZeroOrderHold  SampleTime=model.dt
  h : Scope  NumInputPorts=2
      settings: SampleTime=5/60  ActiveDisplayYMinimum=4.45610108475343  ActiveDisplayYMaximum=7.5358609654106035  DataLoggingVariableName=ScopeData9
  h  M.noise : dspsrcs4/Random Source  SrcType=Gaussian  MinVal=0  MaxVal=1  MeanVal=0  VarVal=noise.M.h.*noise.M.active  RepMode=Not repeatable  rawSeed=78  IsInherit=off  SampTime=model.dt  SampFrame=1  OutComplex=Real  DataType=double  SimulateUsing=Interpreted execution
  l(Q) : Scope
      settings: ActiveDisplayYMinimum=-0.024834753778036393  ActiveDisplayYMaximum=1.1656414366981545  DataLoggingVariableName=ScopeData3
  l(Q_C) : Scope
      settings: ActiveDisplayYMinimum=-0.024032526120106434  ActiveDisplayYMaximum=1.0168626297786216  DataLoggingVariableName=ScopeData11
  wires:
  Saturation2/1 -> Subsystem6/3(T_F), Sum31/2
  Sum8/1 -> Saturation4/1
  Sum3/1 -> Saturation3/1
  Saturation1/1 -> Subsystem6/2(Q_F), Sum27/2
  Q_C M.noise/1 -> Sum4/2
  SS.SP_T/1 -> Sum9/2
  Sum6/1 -> Sum30/2, Gain4/1  "Tm"
  SS.SP_Q_C/1 -> Sum10/1
  F6/1 -> F6_active/1
  Sum11/1 -> Sum1/2
  F6_active/1 -> Sum11/1
  Sum12/1 -> Sum2/2
  Gain21/1 -> E_Q_C/1, Transfer Fcn1/1  "E_Q_C"
  Gain20/1 -> E_T/1, Transfer Fcn/1  "E_T"
  Sum23/1 -> Sum7/2
  Sum20/1 -> Zero-Order Hold7/1, Gain5/1  "hm"
  Subsystem6/3(h) -> Sum20/1
  Clock1/1 -> F12/1(t), To Workspace14/1, Switch/2
  h  M.noise/1 -> Sum20/2
  SS.SP_Q/1 -> Sum17/2
  Q  M.noise/1 -> Sum18/2
  Gc_Q/1 -> Gain13/1, Gv_l(Q)/1
  Gain19/1 -> E_h/1, Transfer Fcn3/1  "E_h"
  Gc_h/1 -> Sum17/1, Gain12/1  "SP_Q'"
  Gain22/1 -> Transfer Fcn2/1, E_Q/1  "E_Q"
  Sum18/1 -> Gain6/1, Zero-Order Hold8/1  "Qm"
  T  M.noise/1 -> Sum6/2
  F7_active/1 -> Sum13/1
  Sum13/1 -> Sum3/2
  Sum15/1 -> Sum8/2
  F10_active/1 -> Sum23/1
  F10/1 -> F10_active/1
  SS.P_CU/1 -> Sum7/1
  SS.T_CF/1 -> Sum8/1
  SS.C_AF/1 -> Sum3/1
  SS.T_F/1 -> Sum2/3
  SS.Q_F/1 -> Sum1/3
  SS.P_CD/1 -> Sum23/2
  SS.lQ_C/1 -> Sum25/1
  Saturation/1 -> l(Q_C)/1, Subsystem2/2(In2)
  SS.P_D/1 -> Sum26/2
  Gain1/1 -> Sqrt1/1
  Sum26/1 -> Sum28/2
  Sum28/1 -> Gain1/1
  SS.P_U/1 -> Sum28/3
  F11_active/1 -> Sum26/1
  SS.LQ/1 -> Sum29/1
  C_A M.noise/1 -> Sum14/2
  Gain2/1 -> To Workspace/1
  Gain3/1 -> To Workspace1/1
  Gain4/1 -> To Workspace2/1
  Gain5/1 -> To Workspace3/1
  Gain6/1 -> To Workspace4/1
  Gain7/1 -> To Workspace5/1
  Gain8/1 -> To Workspace6/1
  Gain9/1 -> To Workspace7/1
  Gain10/1 -> To Workspace8/1
  Gain11/1 -> To Workspace9/1
  Gain12/1 -> To Workspace10/1
  Gain13/1 -> To Workspace11/1
  Gain15/1 -> To Workspace13/1
  Gc_T/1 -> Gain14/1, Sum10/2  "SP_Q'"
  Gain14/1 -> To Workspace12/1
  F12_active/1 -> Switch/1
  F_6/1 -> F_6_active/1
  F_6_active/1 -> Sum11/3
  F3/1(Q_Cm) -> Gain7/1, Zero-Order Hold2/1  "Q_Cm"
  Sum4/1 -> F3/1(1)
  F4/1 -> F4_active/1
  F4_active/1 -> Sum30/1
  F_4/1 -> F_4_active/1
  F_4_active/1 -> Sum30/3
  F7/1 -> F7_active/1
  F_7/1 -> F_7_active/1
  F_7_active/1 -> Sum13/2
  F8_active/1 -> Sum12/1
  F_8_active/1 -> Sum12/2
  F_8/1 -> F_8_active/1
  F8/1 -> F8_active/1
  F_9/1 -> F_9_active/1
  F_9_active/1 -> Sum15/2
  F9_active/1 -> Sum15/1
  F9/1 -> F9_active/1
  F_10/1 -> F_10_active/1
  F_10_active/1 -> Sum23/3
  F_11/1 -> F_11_active/1
  F11/1 -> F11_active/1
  F_11_active/1 -> Sum26/3
  S_1/1 -> S_1_active/1
  S1/1 -> S1_active/1
  S_1_active/1 -> Sum9/3
  S1_active/1 -> Sum9/1
  F12/1(Out1) -> F12_active/1
  Subsystem6/4(C_A) -> Sum14/1
  Sum14/1 -> Scope/1, Gain2/1
  Subsystem6/2(T) -> Sum6/1
  Switch/1 -> Sum11/2
  Sum25/1 -> Saturation/1
  Sum1/1 -> Saturation1/1  "Q_F"
  Sum2/1 -> Saturation2/1  "T_F"
  Saturation3/1 -> Sum32/2, Subsystem6/4(C_AF)
  Saturation4/1 -> Sum33/2, Subsystem6/5(T_CF)
  Sum29/1 -> Saturation5/1
  Gc_Q_C/1 -> Gv_l(Q_C)/1, Gain15/1
  Sqrt1/1 -> Gain16/1
  Sum7/1 -> Gain17/1
  Gain17/1 -> Sqrt2/1
  Sqrt2/1 -> Gain18/1
  Transfer Fcn3/1 -> Gc_h/1
  Transfer Fcn2/1 -> Gc_Q/1
  Transfer Fcn1/1 -> Gc_Q_C/1
  Sum10/1 -> Q_C/2, Sum/1  "SP_Q_C"
  Zero-Order Hold2/1 -> Saturation9/1
  Zero-Order Hold3/1 -> Saturation8/1
  Sum30/1 -> Zero-Order Hold3/1  "Tm"
  Sum9/1 -> T/2, Sum5/1  "SP_T"
  Gain18/1 -> Subsystem2/1(In1)
  Subsystem1/1(Out1) -> Sum18/1, Subsystem6/1(Q)
  Gain16/1 -> Subsystem1/2(In2)
  Saturation5/1 -> Subsystem1/1(In1), l(Q)/1
  Sum17/1 -> Sum16/2, Q/2  "SP_Q"
  SS.SP_h/1 -> h/2, Sum19/2  "SP_h"
  Zero-Order Hold8/1 -> Saturation7/1
  Zero-Order Hold7/1 -> Saturation6/1
  Transfer Fcn/1 -> Gc_T/1
  Saturation6/1 -> Sum19/1, h/1  "hm"
  Saturation8/1 -> Sum5/2, T/1  "Tm"
  Saturation9/1 -> Q_C/1, Sum/2  "Q_Cm"
  Saturation7/1 -> Sum16/1, Q/1  "Qm"
  Subsystem9/1(Out1) -> Sum28/1
  Subsystem2/1(Out1) -> Sum4/1, Subsystem6/6(Q_C)
  Gv_l(Q_C)/1 -> Sum25/2
  Gv_l(Q)/1 -> Sum29/2
  P_D AR.noise/1 -> Subsystem9/1(In1)
  Q_F AR.noise/1 -> Subsystem8/1(In1)
  Subsystem8/1(Out1) -> Sum1/1
  T_F AR.noise/1 -> Subsystem7/1(In1)
  Subsystem7/1(Out1) -> Sum2/1
  Subsystem5/1(Out1) -> Sum3/3
  Subsystem4/1(Out1) -> Sum8/3
  Subsystem3/1(Out1) -> Sum7/3
  P_CU AR.noise/1 -> Subsystem3/1(In1)
  T_CF AR.noise/1 -> Subsystem4/1(In1)
  C_AF AR.noise/1 -> Subsystem5/1(In1)
  T_C  M.noise/1 -> Sum21/2
  Subsystem6/1(T_C) -> Sum21/1
  Sum21/1 -> Gain3/1  "Tm"
  Q_F M.noise/1 -> Sum27/1
  Sum27/1 -> Gain8/1
  T_F M.noise/1 -> Sum31/1
  Sum31/1 -> Gain9/1
  C_AF M.noise/1 -> Sum32/1
  Sum32/1 -> Gain10/1
  Sum33/1 -> Gain11/1
  T_CF M.noise/1 -> Sum33/1
  Sum5/1 -> Gain20/1
  Sum19/1 -> Gain19/1
  Sum/1 -> Gain21/1
  Sum16/1 -> Gain22/1

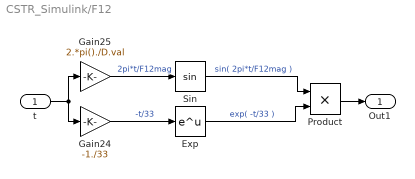
== system CSTR_Simulink/F12 ==
  t : Inport
  Exp : Math
  Gain24 : Gain  Gain=-1./33
  Gain25 : Gain  Gain=2.*pi()./D.val
  Product : Product
  Sin : Trigonometry
  Out1 : Outport
  wires:
  Gain25/1 -> Sin/1  "2pi*t/F12mag"
  Product/1 -> Out1/1
  t/1 -> Gain24/1, Gain25/1
  Gain24/1 -> Exp/1  "-t/33"
  Exp/1 -> Product/2  "exp( -t/33 )"
  Sin/1 -> Product/1  "sin( 2pi*t/F12mag )"

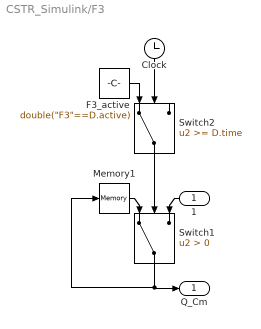
== system CSTR_Simulink/F3 ==
  1 : Inport
  Clock : Clock
  F3_active : Constant  Value="double(\"F3\"==D.active)"
  Memory1 : Memory  InheritSampleTime=on
  Switch1 : Switch  Criteria=u2 > Threshold  SaturateOnIntegerOverflow=off  InputSameDT=off
  Switch2 : Switch  Threshold=D.time  SaturateOnIntegerOverflow=off  InputSameDT=off
  Q_Cm : Outport
  wires:
  Clock/1 -> Switch2/2
  Switch2/1 -> Switch1/2
  Memory1/1 -> Switch1/1
  1/1 -> Switch1/3
  F3_active/1 -> Switch2/1
  Switch1/1 -> Q_Cm/1, Memory1/1

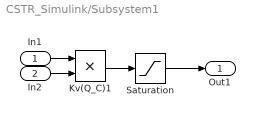
== system CSTR_Simulink/Subsystem1 ==
  In1 : Inport
  In2 : Inport  Port=2
  Kv(Q_C)1 : Product
  Saturation : Saturate  UpperLimit=inf  LowerLimit=0
  Out1 : Outport
  wires:
  In2/1 -> Kv(Q_C)1/2
  Kv(Q_C)1/1 -> Saturation/1
  In1/1 -> Kv(Q_C)1/1
  Saturation/1 -> Out1/1

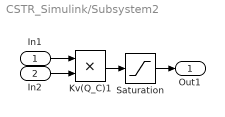
== system CSTR_Simulink/Subsystem2 ==
  In1 : Inport
  In2 : Inport  Port=2
  Kv(Q_C)1 : Product
  Saturation : Saturate  UpperLimit=inf  LowerLimit=0
  Out1 : Outport
  wires:
  In2/1 -> Kv(Q_C)1/2
  Kv(Q_C)1/1 -> Saturation/1
  In1/1 -> Kv(Q_C)1/1
  Saturation/1 -> Out1/1

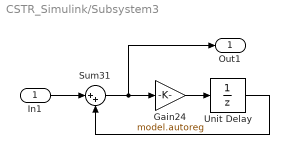
== system CSTR_Simulink/Subsystem3 ==
  In1 : Inport
  Gain24 : Gain  Gain=model.autoreg
  Sum31 : Sum  Inputs=|++
  Unit Delay : UnitDelay  SampleTime=-1
  Out1 : Outport
  wires:
  In1/1 -> Sum31/1
  Sum31/1 -> Gain24/1, Out1/1
  Unit Delay/1 -> Sum31/2
  Gain24/1 -> Unit Delay/1

== system CSTR_Simulink/Subsystem4 ==
  In1 : Inport
  Gain24 : Gain  Gain=model.autoreg
  Sum31 : Sum  Inputs=|++
  Unit Delay : UnitDelay  SampleTime=-1
  Out1 : Outport
  wires:
  In1/1 -> Sum31/1
  Sum31/1 -> Gain24/1, Out1/1
  Unit Delay/1 -> Sum31/2
  Gain24/1 -> Unit Delay/1

== system CSTR_Simulink/Subsystem5 ==
  In1 : Inport
  Gain24 : Gain  Gain=model.autoreg
  Sum31 : Sum  Inputs=|++
  Unit Delay : UnitDelay  SampleTime=-1
  Out1 : Outport
  wires:
  In1/1 -> Sum31/1
  Sum31/1 -> Gain24/1, Out1/1
  Unit Delay/1 -> Sum31/2
  Gain24/1 -> Unit Delay/1

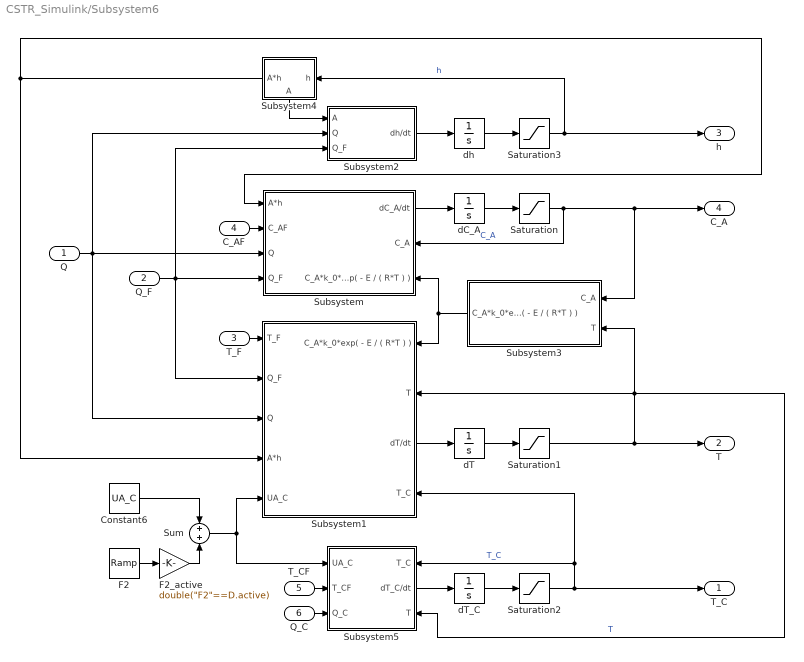
== system CSTR_Simulink/Subsystem6 ==
  Q : Inport
  Q_F : Inport  Port=2
  T_F : Inport  Port=3
  C_AF : Inport  Port=4
  T_CF : Inport  Port=5
  Q_C : Inport  Port=6
  Constant6 : Constant  Value=UA_C
  F2 : simulink/Sources/Ramp  slope=D.val  start=D.time  InitialOutput=0
  F2_active : Gain  Gain="double(\"F2\"==D.active)"
  Saturation : Saturate  UpperLimit=inf  LowerLimit=0
  Saturation1 : Saturate  UpperLimit=inf  LowerLimit=0
  Saturation2 : Saturate  UpperLimit=inf  LowerLimit=0
  Saturation3 : Saturate  UpperLimit=inf  LowerLimit=0.01
  Subsystem : Subsystem
      settings: PortSchema="{\"entries\":[{\"content\":{\"sides\":[{\"content\":{\"connectorIds\":[\"In1\",\"In2\",\"In3\",\"In4\"]},\"type\":\"ConnectorPlacement.EquallySpacedRectSide\",\"uuid\":\"0b1324c4-900f-4f94-b577-5ef39242d251\"},{\"content\":{\"connectorIds\":[\"Out1\",\"In5\",\"In6\"],\"side\":\"RIGHT\"},\"type\":\"ConnectorPlacement.EquallySpacedRectSide\",\"uuid\":\"04b59dc5-7050-4ee2-b870-ec2358d44a74\"},{\"content\":{\"side\":\"TOP\"},\"type\":\"ConnectorPlacement.EquallySpacedRectSide\",\"uuid\":\"6b691fdb-a0e1-4607-aa3c-ba54b3dd7d53\"}]},\"type\":\"ConnectorPlacement.EquallySpacedConnector\",\"uuid\":\"86f059ce-7a39-4ec5-aac4-fd7ad5891f3b\"}],\"packageUris\":[\"http://schema.mathworks.com/mf0/Connector/R2020b\"],\"version\":\"1.0\"}"
  Subsystem1 : Subsystem
      settings: PortSchema="{\"entries\":[{\"content\":{\"sides\":[{\"content\":{\"connectorIds\":[\"In1\",\"In2\",\"In3\",\"In4\",\"In5\"]},\"type\":\"ConnectorPlacement.EquallySpacedRectSide\",\"uuid\":\"aa888c54-b043-45b1-a37f-b543a5d68719\"},{\"content\":{\"connectorIds\":[\"In6\",\"In7\",\"Out1\",\"In8\"],\"side\":\"RIGHT\"},\"type\":\"ConnectorPlacement.EquallySpacedRectSide\",\"uuid\":\"a33c504f-62aa-4b43-9fb0-649efe901050\"},{\"content\":{\"side\":\"TOP\"},\"type\":\"ConnectorPlacement.EquallySpacedRectSide\",\"uuid\":\"74edb8fc-d4a6-43b3-ba63-608d609d4ced\"}]},\"type\":\"ConnectorPlacement.EquallySpacedConnector\",\"uuid\":\"90fa1944-24fb-42b7-99b7-30ce6c9cbe76\"}],\"packageUris\":[\"http://schema.mathworks.com/mf0/Connector/R2020b\"],\"version\":\"1.0\"}"
  Subsystem2 : Subsystem
  Subsystem3 : Subsystem
  Subsystem4 : Subsystem
      settings: PortSchema="{\"entries\":[{\"content\":{\"sides\":[{\"content\":{\"connectorIds\":[\"Out2\"]},\"type\":\"ConnectorPlacement.EquallySpacedRectSide\",\"uuid\":\"fe5db84a-3abb-42c1-9cae-e7aa606272c9\"},{\"content\":{\"connectorIds\":[\"In1\"],\"side\":\"RIGHT\"},\"type\":\"ConnectorPlacement.EquallySpacedRectSide\",\"uuid\":\"aa77bc2b-e653-43f2-b429-1f04fd46988f\"},{\"content\":{\"side\":\"TOP\"},\"type\":\"ConnectorPlacement.EquallySpacedRectSide\",\"uuid\":\"65d2b64b-1f2d-43d9-a93e-6f3060fc3d1d\"},{\"content\":{\"connectorIds\":[\"Out1\"],\"side\":\"BOTTOM\"},\"type\":\"ConnectorPlacement.EquallySpacedRectSide\",\"uuid\":\"ae6f78b6-8207-4b67-b1de-eeea5ebdd0f9\"}]},\"type\":\"ConnectorPlacement.EquallySpacedConnector\",\"uuid\":\"b79708e3-556f-413c-9a44-b43c1290d1fc\"}],\"packageUris\":[\"http://schema.mathworks.com/mf0/Connector/R2020b\"],\"version\":\"1.0\"}"
  Subsystem5 : Subsystem
      settings: PortSchema="{\"entries\":[{\"content\":{\"sides\":[{\"content\":{\"connectorIds\":[\"In1\",\"In2\",\"In3\"]},\"type\":\"ConnectorPlacement.EquallySpacedRectSide\",\"uuid\":\"44147885-6c11-496b-8977-f00f34833e36\"},{\"content\":{\"connectorIds\":[\"In4\",\"Out1\",\"In5\"],\"side\":\"RIGHT\"},\"type\":\"ConnectorPlacement.EquallySpacedRectSide\",\"uuid\":\"19e22ec1-6a70-4dbd-8ccb-a3fc5fe153c3\"},{\"content\":{\"side\":\"TOP\"},\"type\":\"ConnectorPlacement.EquallySpacedRectSide\",\"uuid\":\"f8ef5438-1537-4889-9469-444b48567eee\"}]},\"type\":\"ConnectorPlacement.EquallySpacedConnector\",\"uuid\":\"42cc88af-1ffd-4590-8c64-1c0228614b8b\"}],\"packageUris\":[\"http://schema.mathworks.com/mf0/Connector/R2020b\"],\"version\":\"1.0\"}"
  Sum : Sum  Inputs=+|+
  dC_A : Integrator  InitialCondition=SS.C_A
  dT : Integrator  InitialCondition=SS.T
  dT_C : Integrator  InitialCondition=SS.T_C
  dh : Integrator  InitialCondition=SS.h
  T_C : Outport
  T : Outport  Port=2
  h : Outport  Port=3
  C_A : Outport  Port=4
  wires:
  Subsystem5/1(dT_C/dt) -> dT_C/1
  Sum/1 -> Subsystem5/1(UA_C), Subsystem1/5(UA_C)
  Saturation/1 -> Subsystem/5(C_A), C_A/1, Subsystem3/1(C_A)  "C_A"
  Subsystem4/1(A) -> Subsystem2/1(A)
  Subsystem4/2(A*h) -> Subsystem1/4(A*h), Subsystem/1(A*h)
  Saturation3/1 -> h/1, Subsystem4/1(h)  "h"
  Q_F/1 -> Subsystem1/2(Q_F), Subsystem/4(Q_F), Subsystem2/3(Q_F)
  Saturation1/1 -> T/1, Subsystem1/7(T), Subsystem5/5(T), Subsystem3/2(T)  "T"
  Subsystem1/1(dT/dt) -> dT/1
  Saturation2/1 -> T_C/1, Subsystem5/4(T_C), Subsystem1/8(T_C)  "T_C"
  Q/1 -> Subsystem1/3(Q), Subsystem2/2(Q), Subsystem/3(Q)
  C_AF/1 -> Subsystem/2(C_AF)
  Subsystem/1(dC_A/dt) -> dC_A/1
  Subsystem3/1(C_A*k_0*exp( - E / ( R*T ) )) -> Subsystem/6(C_A*k_0*exp( - E / ( R*T ) )), Subsystem1/6(C_A*k_0*exp( - E / ( R*T ) ))
  T_CF/1 -> Subsystem5/2(T_CF)
  T_F/1 -> Subsystem1/1(T_F)
  Subsystem2/1(dh/dt) -> dh/1
  Q_C/1 -> Subsystem5/3(Q_C)
  F2/1 -> F2_active/1
  F2_active/1 -> Sum/2
  Constant6/1 -> Sum/1
  dC_A/1 -> Saturation/1
  dT/1 -> Saturation1/1
  dT_C/1 -> Saturation2/1
  dh/1 -> Saturation3/1

== system CSTR_Simulink/Subsystem7 ==
  In1 : Inport
  Gain24 : Gain  Gain=model.autoreg
  Sum31 : Sum  Inputs=|++
  Unit Delay : UnitDelay  SampleTime=-1
  Out1 : Outport
  wires:
  In1/1 -> Sum31/1
  Sum31/1 -> Gain24/1, Out1/1
  Unit Delay/1 -> Sum31/2
  Gain24/1 -> Unit Delay/1

== system CSTR_Simulink/Subsystem8 ==
  In1 : Inport
  Gain24 : Gain  Gain=model.autoreg
  Sum31 : Sum  Inputs=|++
  Unit Delay : UnitDelay  SampleTime=-1
  Out1 : Outport
  wires:
  In1/1 -> Sum31/1
  Sum31/1 -> Gain24/1, Out1/1
  Unit Delay/1 -> Sum31/2
  Gain24/1 -> Unit Delay/1

== system CSTR_Simulink/Subsystem9 ==
  In1 : Inport
  Gain24 : Gain  Gain=model.autoreg
  Sum31 : Sum  Inputs=|++
  Unit Delay : UnitDelay  SampleTime=-1
  Out1 : Outport
  wires:
  Sum31/1 -> Gain24/1, Out1/1
  Unit Delay/1 -> Sum31/2
  Gain24/1 -> Unit Delay/1
  In1/1 -> Sum31/1

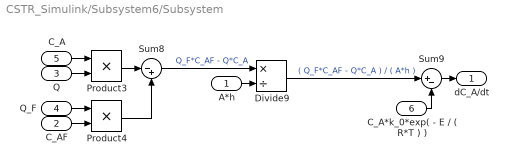
== system CSTR_Simulink/Subsystem6/Subsystem ==
  A*h : Inport
  C_AF : Inport  Port=2
  Q : Inport  Port=3
  Q_F : Inport  Port=4
  C_A : Inport  Port=5
  C_A*k_0*exp( - E / ( R*T ) ) : Inport  Port=6
  Divide9 : Product  Inputs=*/
  Product3 : Product
  Product4 : Product
  Sum8 : Sum  Inputs=|-+
  Sum9 : Sum  Inputs=|+-
  dC_A/dt : Outport
  wires:
  Q/1 -> Product3/2
  Product4/1 -> Sum8/2
  Product3/1 -> Sum8/1
  C_AF/1 -> Product4/2
  Divide9/1 -> Sum9/1  "( Q_F*C_AF - Q*C_A ) / ( A*h )"
  C_A*k_0*exp( - E / ( R*T ) )/1 -> Sum9/2
  A*h/1 -> Divide9/2
  Sum8/1 -> Divide9/1  "Q_F*C_AF - Q*C_A"
  Sum9/1 -> dC_A/dt/1
  C_A/1 -> Product3/1
  Q_F/1 -> Product4/1

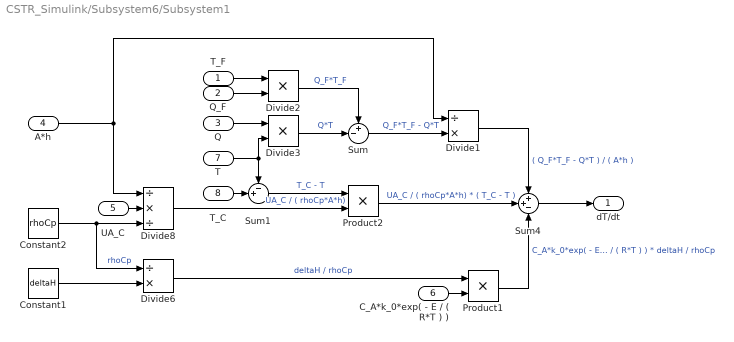
== system CSTR_Simulink/Subsystem6/Subsystem1 ==
  T_F : Inport  PortDimensions=1
  Q_F : Inport  Port=2  PortDimensions=1
  Q : Inport  Port=3  PortDimensions=1
  A*h : Inport  Port=4  PortDimensions=1
  UA_C : Inport  Port=5  PortDimensions=1
  C_A*k_0*exp( - E / ( R*T ) ) : Inport  Port=6  PortDimensions=1
  T : Inport  Port=7  PortDimensions=1
  T_C : Inport  Port=8  PortDimensions=1
  Constant1 : Constant  Value=deltaH
  Constant2 : Constant  Value=rhoCp
  Divide1 : Product  Inputs=/*
  Divide2 : Product  Inputs=**
  Divide3 : Product  Inputs=**
  Divide6 : Product  Inputs=/*
  Divide8 : Product  Inputs=/*/
  Product1 : Product
  Product2 : Product
  Sum : Sum  Inputs=+-|
  Sum1 : Sum  Inputs=-+|
  Sum4 : Sum  Inputs=++-
  dT/dt : Outport
  wires:
  Divide8/1 -> Product2/2  "UA_C / ( rhoCp*A*h)"
  Product1/1 -> Sum4/3  "C_A*k_0*exp( - E / ( R*T ) ) * deltaH / rhoCp"
  Product2/1 -> Sum4/2  "UA_C / ( rhoCp*A*h) * ( T_C - T )"
  Divide3/1 -> Sum/2  "Q*T"
  T/1 -> Divide3/2, Sum1/1
  Divide1/1 -> Sum4/1  "( Q_F*T_F - Q*T ) / ( A*h )"
  Divide2/1 -> Sum/1  "Q_F*T_F"
  Sum/1 -> Divide1/2  "Q_F*T_F - Q*T"
  A*h/1 -> Divide1/1, Divide8/1
  UA_C/1 -> Divide8/2
  Sum4/1 -> dT/dt/1
  Q/1 -> Divide3/1
  T_F/1 -> Divide2/1
  T_C/1 -> Sum1/2
  Q_F/1 -> Divide2/2
  C_A*k_0*exp( - E / ( R*T ) )/1 -> Product1/2
  Constant1/1 -> Divide6/2
  Divide6/1 -> Product1/1  "deltaH / rhoCp"
  Constant2/1 -> Divide8/3, Divide6/1  "rhoCp"
  Sum1/1 -> Product2/1  "T_C - T"

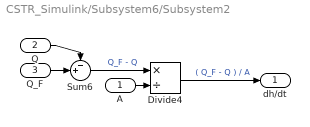
== system CSTR_Simulink/Subsystem6/Subsystem2 ==
  A : Inport
  Q : Inport  Port=2
  Q_F : Inport  Port=3
  Divide4 : Product  Inputs=*/
  Sum6 : Sum  Inputs=-+|
  dh/dt : Outport
  wires:
  Divide4/1 -> dh/dt/1  "( Q_F - Q ) / A"
  Sum6/1 -> Divide4/1  "Q_F - Q"
  Q_F/1 -> Sum6/2
  A/1 -> Divide4/2
  Q/1 -> Sum6/1

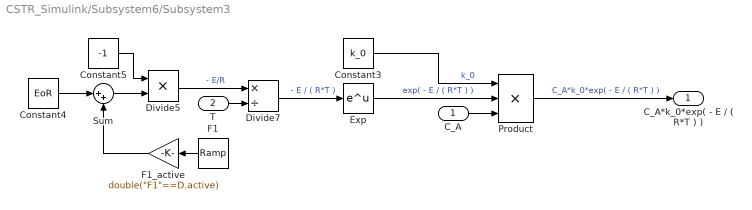
== system CSTR_Simulink/Subsystem6/Subsystem3 ==
  C_A : Inport
  T : Inport  Port=2
  Constant3 : Constant  Value=k_0
  Constant4 : Constant  Value=EoR
  Constant5 : Constant  Value=-1
  Divide5 : Product  Inputs=**
  Divide7 : Product  Inputs=*/
  Exp : Math
  F1 : simulink/Sources/Ramp  slope=D.val  start=D.time  InitialOutput=0
  F1_active : Gain  Gain="double(\"F1\"==D.active)"
  Product : Product  Inputs=3
  Sum : Sum  Inputs=|++
  C_A*k_0*exp( - E / ( R*T ) ) : Outport
  wires:
  Exp/1 -> Product/2  "exp( - E / ( R*T ) )"
  Divide7/1 -> Exp/1  "- E / ( R*T )"
  T/1 -> Divide7/2
  Constant5/1 -> Divide5/1
  Constant3/1 -> Product/1  "k_0"
  Constant4/1 -> Sum/1
  Divide5/1 -> Divide7/1  "- E/R"
  Product/1 -> C_A*k_0*exp( - E / ( R*T ) )/1  "C_A*k_0*exp( - E / ( R*T ) )"
  C_A/1 -> Product/3
  Sum/1 -> Divide5/2
  F1/1 -> F1_active/1
  F1_active/1 -> Sum/2

== system CSTR_Simulink/Subsystem6/Subsystem4 ==
  h : Inport
  Constant : Constant  Value=A
  Divide : Product  Inputs=**
  A : Outport
  A*h : Outport  Port=2
  wires:
  Divide/1 -> A*h/1
  Constant/1 -> Divide/2, A/1
  h/1 -> Divide/1
